simulink model "Q5_2_1"  (R2023b)
settings: Solver=ode45  StartTime=0.0  StopTime=15.0  RelTol=1e-3
settings Model: Creator=Arshia  LastModifiedBy=Arshia

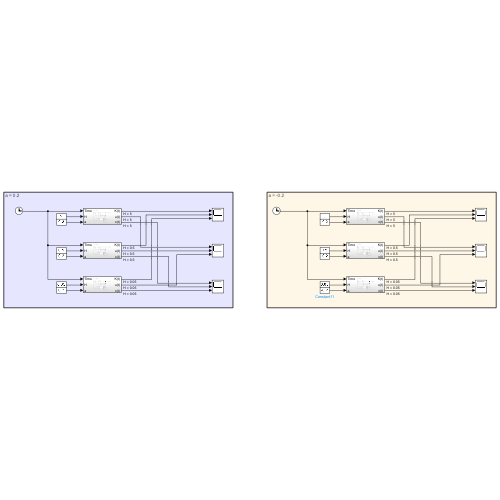
[thumbnail: Simulink's stored preview of the top-level diagram]
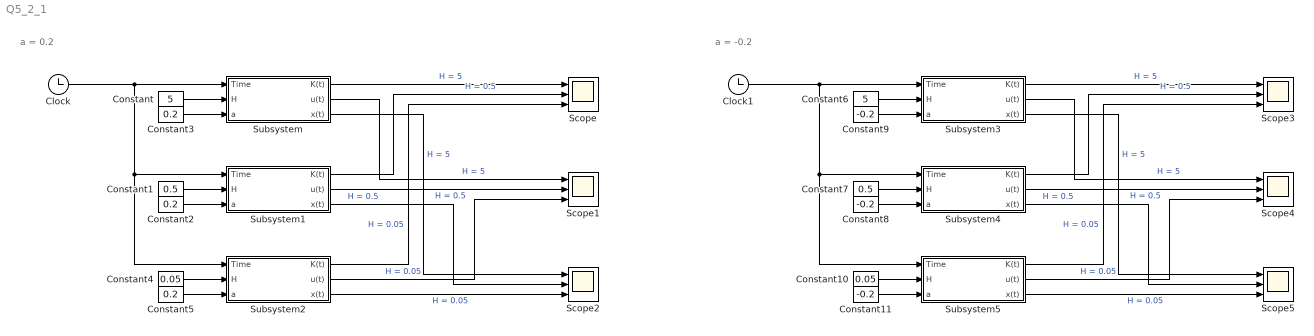
== system Q5_2_1 ==
  note: a = 0.2
  note: a = -0.2
  Clock : Clock
  Clock1 : Clock
  Constant : Constant  Value=5
  Constant1 : Constant  Value=0.5
  Constant10 : Constant  Value=0.05
  Constant11 : Constant  Value=-0.2
  Constant2 : Constant  Value=0.2
  Constant3 : Constant  Value=0.2
  Constant4 : Constant  Value=0.05
  Constant5 : Constant  Value=0.2
  Constant6 : Constant  Value=5
  Constant7 : Constant  Value=0.5
  Constant8 : Constant  Value=-0.2
  Constant9 : Constant  Value=-0.2
  Scope{,1..5} (6 alike) : Scope  NumInputPorts=3
  Subsystem : Subsystem
  Subsystem1 : Subsystem
  Subsystem2 : Subsystem
  Subsystem3 : Subsystem
  Subsystem4 : Subsystem
  Subsystem5 : Subsystem
  wires:
  Constant/1 -> Subsystem/2(H)
  Constant3/1 -> Subsystem/3(a)
  Constant2/1 -> Subsystem1/3(a)
  Constant1/1 -> Subsystem1/2(H)
  Constant5/1 -> Subsystem2/3(a)
  Constant4/1 -> Subsystem2/2(H)
  Subsystem/1(K(t)) -> Scope/1  "H = 5"
  Subsystem1/1(K(t)) -> Scope/2  "H = 0.5"
  Subsystem2/1(K(t)) -> Scope/3  "H = 0.05"
  Subsystem/2(u(t)) -> Scope1/1  "H = 5"
  Subsystem1/2(u(t)) -> Scope1/2  "H = 0.5"
  Subsystem2/2(u(t)) -> Scope1/3  "H = 0.05"
  Subsystem/3(x(t)) -> Scope2/1  "H = 5"
  Subsystem1/3(x(t)) -> Scope2/2  "H = 0.5"
  Subsystem2/3(x(t)) -> Scope2/3  "H = 0.05"
  Subsystem4/2(u(t)) -> Scope4/2  "H = 0.5"
  Subsystem3/1(K(t)) -> Scope3/1  "H = 5"
  Subsystem4/1(K(t)) -> Scope3/2  "H = 0.5"
  Constant9/1 -> Subsystem3/3(a)
  Subsystem5/3(x(t)) -> Scope5/3  "H = 0.05"
  Subsystem5/1(K(t)) -> Scope3/3  "H = 0.05"
  Constant10/1 -> Subsystem5/2(H)
  Constant11/1 -> Subsystem5/3(a)
  Constant6/1 -> Subsystem3/2(H)
  Clock/1 -> Subsystem2/1(Time), Subsystem1/1(Time), Subsystem/1(Time)
  Subsystem3/2(u(t)) -> Scope4/1  "H = 5"
  Subsystem4/3(x(t)) -> Scope5/2  "H = 0.5"
  Constant7/1 -> Subsystem4/2(H)
  Subsystem3/3(x(t)) -> Scope5/1  "H = 5"
  Subsystem5/2(u(t)) -> Scope4/3  "H = 0.05"
  Constant8/1 -> Subsystem4/3(a)
  Clock1/1 -> Subsystem3/1(Time), Subsystem5/1(Time), Subsystem4/1(Time)

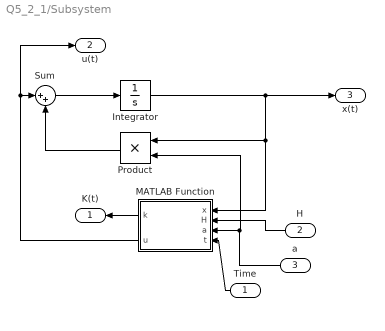
== system Q5_2_1/Subsystem ==
  Time : Inport
  H : Inport  Port=2
  a : Inport  Port=3
  Integrator : Integrator  InitialCondition=5
  MATLAB Function : MATLAB Function  TreatAsAtomicUnit=on
  Product : Product
  Sum : Sum  Inputs=|++
  K(t) : Outport
  u(t) : Outport  Port=2
  x(t) : Outport  Port=3
  wires:
  Time/1 -> MATLAB Function/4(t)
  MATLAB Function/2(u) -> Sum/1, u(t)/1
  Sum/1 -> Integrator/1
  Integrator/1 -> MATLAB Function/1(x), Product/1, x(t)/1
  H/1 -> MATLAB Function/2(H)
  Product/1 -> Sum/2
  MATLAB Function/1(k) -> K(t)/1
  a/1 -> Product/2, MATLAB Function/3(a)

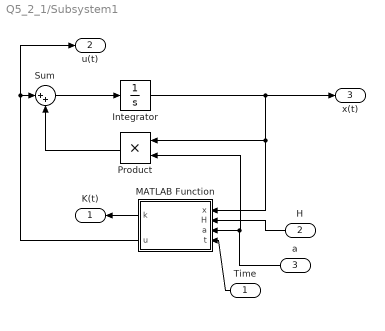
== system Q5_2_1/Subsystem1 ==
  Time : Inport
  H : Inport  Port=2
  a : Inport  Port=3
  Integrator : Integrator  InitialCondition=5
  MATLAB Function : MATLAB Function  TreatAsAtomicUnit=on
  Product : Product
  Sum : Sum  Inputs=|++
  K(t) : Outport
  u(t) : Outport  Port=2
  x(t) : Outport  Port=3
  wires:
  Time/1 -> MATLAB Function/4(t)
  MATLAB Function/2(u) -> Sum/1, u(t)/1
  Sum/1 -> Integrator/1
  Integrator/1 -> MATLAB Function/1(x), Product/1, x(t)/1
  H/1 -> MATLAB Function/2(H)
  Product/1 -> Sum/2
  MATLAB Function/1(k) -> K(t)/1
  a/1 -> Product/2, MATLAB Function/3(a)

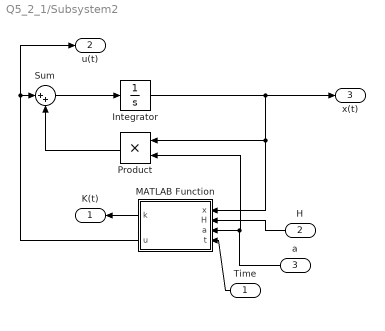
== system Q5_2_1/Subsystem2 ==
  Time : Inport
  H : Inport  Port=2
  a : Inport  Port=3
  Integrator : Integrator  InitialCondition=5
  MATLAB Function : MATLAB Function  TreatAsAtomicUnit=on
  Product : Product
  Sum : Sum  Inputs=|++
  K(t) : Outport
  u(t) : Outport  Port=2
  x(t) : Outport  Port=3
  wires:
  Time/1 -> MATLAB Function/4(t)
  MATLAB Function/2(u) -> Sum/1, u(t)/1
  Sum/1 -> Integrator/1
  Integrator/1 -> MATLAB Function/1(x), Product/1, x(t)/1
  H/1 -> MATLAB Function/2(H)
  Product/1 -> Sum/2
  MATLAB Function/1(k) -> K(t)/1
  a/1 -> Product/2, MATLAB Function/3(a)

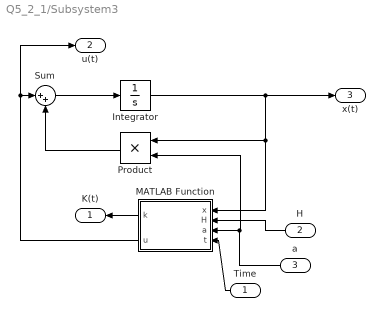
== system Q5_2_1/Subsystem3 ==
  Time : Inport
  H : Inport  Port=2
  a : Inport  Port=3
  Integrator : Integrator  InitialCondition=5
  MATLAB Function : MATLAB Function  TreatAsAtomicUnit=on
  Product : Product
  Sum : Sum  Inputs=|++
  K(t) : Outport
  u(t) : Outport  Port=2
  x(t) : Outport  Port=3
  wires:
  Time/1 -> MATLAB Function/4(t)
  MATLAB Function/2(u) -> Sum/1, u(t)/1
  Sum/1 -> Integrator/1
  Integrator/1 -> MATLAB Function/1(x), Product/1, x(t)/1
  H/1 -> MATLAB Function/2(H)
  Product/1 -> Sum/2
  MATLAB Function/1(k) -> K(t)/1
  a/1 -> Product/2, MATLAB Function/3(a)

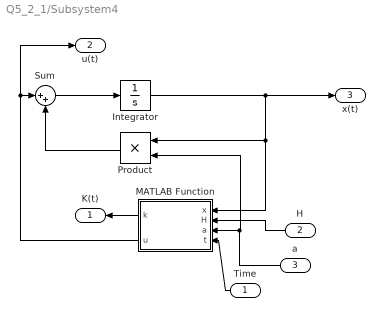
== system Q5_2_1/Subsystem4 ==
  Time : Inport
  H : Inport  Port=2
  a : Inport  Port=3
  Integrator : Integrator  InitialCondition=5
  MATLAB Function : MATLAB Function  TreatAsAtomicUnit=on
  Product : Product
  Sum : Sum  Inputs=|++
  K(t) : Outport
  u(t) : Outport  Port=2
  x(t) : Outport  Port=3
  wires:
  Time/1 -> MATLAB Function/4(t)
  MATLAB Function/2(u) -> Sum/1, u(t)/1
  Sum/1 -> Integrator/1
  Integrator/1 -> MATLAB Function/1(x), Product/1, x(t)/1
  H/1 -> MATLAB Function/2(H)
  Product/1 -> Sum/2
  MATLAB Function/1(k) -> K(t)/1
  a/1 -> Product/2, MATLAB Function/3(a)

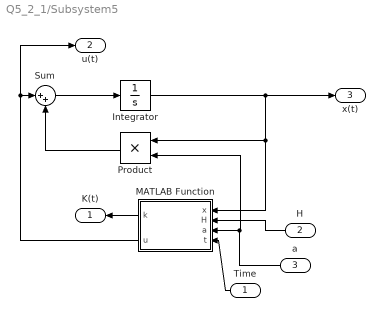
== system Q5_2_1/Subsystem5 ==
  Time : Inport
  H : Inport  Port=2
  a : Inport  Port=3
  Integrator : Integrator  InitialCondition=5
  MATLAB Function : MATLAB Function  TreatAsAtomicUnit=on
  Product : Product
  Sum : Sum  Inputs=|++
  K(t) : Outport
  u(t) : Outport  Port=2
  x(t) : Outport  Port=3
  wires:
  Time/1 -> MATLAB Function/4(t)
  MATLAB Function/2(u) -> Sum/1, u(t)/1
  Sum/1 -> Integrator/1
  Integrator/1 -> MATLAB Function/1(x), Product/1, x(t)/1
  H/1 -> MATLAB Function/2(H)
  Product/1 -> Sum/2
  MATLAB Function/1(k) -> K(t)/1
  a/1 -> Product/2, MATLAB Function/3(a)

== matlab function Q5_2_1/Subsystem1/MATLAB Function ==
  data: x input; k output; H input; a input; t input; u output
function [k,u]= myfcn(x,H,a,t)
k=(pinv(exp(-a*(15-t))-(H/a)*(exp(-a*(15-t))-exp(a*(15-t))))*(H*exp(a*(15-t))));
u=-2*k*x;

== matlab function Q5_2_1/Subsystem/MATLAB Function ==
  data: x input; k output; H input; a input; t input; u output
function [k,u]= myfcn(x,H,a,t)
k=(pinv(exp(-a*(15-t))-(H/a)*(exp(-a*(15-t))-exp(a*(15-t))))*(H*exp(a*(15-t))));
u=-2*k*x;

== matlab function Q5_2_1/Subsystem2/MATLAB Function ==
  data: x input; k output; H input; a input; t input; u output
function [k,u]= myfcn(x,H,a,t)
k=(pinv(exp(-a*(15-t))-(H/a)*(exp(-a*(15-t))-exp(a*(15-t))))*(H*exp(a*(15-t))));
u=-2*k*x;

== matlab function Q5_2_1/Subsystem3/MATLAB Function ==
  data: x input; k output; H input; a input; t input; u output
function [k,u]= myfcn(x,H,a,t)
k=(pinv(exp(-a*(15-t))-(H/a)*(exp(-a*(15-t))-exp(a*(15-t))))*(H*exp(a*(15-t))));
u=-2*k*x;

== matlab function Q5_2_1/Subsystem4/MATLAB Function ==
  data: x input; k output; H input; a input; t input; u output
function [k,u]= myfcn(x,H,a,t)
k=(pinv(exp(-a*(15-t))-(H/a)*(exp(-a*(15-t))-exp(a*(15-t))))*(H*exp(a*(15-t))));
u=-2*k*x;

== matlab function Q5_2_1/Subsystem5/MATLAB Function ==
  data: x input; k output; H input; a input; t input; u output
function [k,u]= myfcn(x,H,a,t)
k=(pinv(exp(-a*(15-t))-(H/a)*(exp(-a*(15-t))-exp(a*(15-t))))*(H*exp(a*(15-t))));
u=-2*k*x;
